simulink model "EV6_LUT_FourWheel_EV6Battery77p4kWh_PowerCorrected"  (R2024a)
settings: Solver=ode4  StartTime=0  StopTime=60  FixedStep=0.001  RelTol=1e-3
PreLoadFcn:
  | VSS_BICYCLE=Simulink.Variant('Dual=0');
  | VSS_DUAL=Simulink.Variant('Dual=1');
  | Dual=1;
  | load('DriveCycle2.mat')
PostLoadFcn:
  | if any(exist('dsrtsu_mdlpostloadfcn', 'file') ~= 0), dsrtsu_mdlpostloadfcn('Execute', bdroot); end
InitFcn:
  | , if any(exist('rtifpga_mdlclblib', 'file') ~= 0), rtifpga_mdlclblib('Init', bdroot); end,
  | , if any(exist('dsmpb_private', 'file') ~= 0), dsmpb_private('dsmpb_mdlclblib', 'Init', bdroot); end,
  | load('DriveCycle2.mat')
model workspace (MAT data in the model file):
  DiffRatio = 10.65
  EV6_2023_BattBranchCapacity_Ah = 55.5236728838
  EV6_2023_BattEnergy_kWh = 77.4
  EV6_2023_BattNominalVoltage_V = 697
  EV6_2023_BattNumCellsParallel = 2
  EV6_2023_BattNumCellsSeries = 192
  EV6_2023_BattOpenVoltCapBpts = [0 0.1 0.2 0.3 0.4 0.5 0.6 0.7 0.8 0.9 1]
  EV6_2023_BattOpenVoltTbl = [2.96762142548 3.40364281191 3.47417488548 3.54470541822 3.61523441014 3.68576186124 3.75628777151 3.82681214095 3.94527005036 4.07101207308 4.2120755254]
  EV6_2023_BattPackCapacity_Ah = 111.047345768
  EV6_2023_BattResistSocBpts = [0 0.2 0.4 0.6 0.8 1]
  EV6_2023_BattResistTbl = [0.0163620057716 0.0118174152018 0.00807187352333 0.00375663957972 0.00266904525531 0.00103635901355 0.0019014404175 0.0172368903217 0.0121226074867 0.00758541551769 0.00474065349228 0.00337561163613 ... (42 elements, 7x6)]
  EV6_2023_BattResistTempBpts = [243.1 253.1 263.1 273.1 283.1 298.1 313.1]
  EV6_2023_InitialPackOCV_V = 726.471714233
  EV6_2023_InitialSOC = 0.638878863672
  EV6_BattCellCapacity_Ah = 60.3
  EV6_BattInitialSOC = 0.638878863672
  EV6_BattOCV_Cell_V = [2.96762142548 3.40364281191 3.47417488548 3.54470541822 3.61523441014 3.68576186124 3.75628777151 3.82681214095 3.94527005036 4.07101207308 4.2120755254]
  EV6_BattOCV_SOC = [0 0.1 0.2 0.3 0.4 0.5 0.6 0.7 0.8 0.9 1]
  EV6_BattPackCapacity_Ah = 120.6
  EV6_BattParallelCells = 2
  EV6_BattResistanceSOC = [0 0.2 0.4 0.6 0.8 1]
  EV6_BattResistanceTable_Ohm = [0.0163620057716 0.0118174152018 0.00807187352333 0.00375663957972 0.00266904525531 0.00103635901355 0.0019014404175 0.0172368903217 0.0121226074867 0.00758541551769 0.00474065349228 0.00337561163613 ... (42 elements, 7x6)]
  EV6_BattResistanceTemp_K = [243.1 253.1 263.1 273.1 283.1 298.1 313.1]
  EV6_BattSeriesCells = 192
  EV6_FinalDriveRatio = 10.65
  EV6_TargetPackResistance_Ohm = 0.132763804608
  Gas = 0.383333333333
undefined symbols (not defined in the file): accel_bp_mps2, AccelCmd, ActTqLF_Nm_, ActTqLR_Nm_, ActTqRF_Nm_, ActTqRR_Nm_, BattChargeLimitMaxPwr, BattChargeLimitSocBpts, BattChargeLimitTbl, BattDischargeLimitSocBpts, BattDischargeLimitTbl, BattDischargeMaxPwr, BrakeMaxPrs, BrakeMaxTrq, ChassisDistCg2FrontAxle, ChassisDistCg2RearAxle, ChassisVehMass, CltchCmd, CoastDown, DecelCmd, DiscIntNeverNeededParam, EnvGravCnst, EnvPrs, EnvTemp, EV6_RegenTorqueGain, EV6_TractionTorqueGain, front_share_regen_3d, front_share_traction_3d, FuelSpecificGrav, GearCmd, h, InitStates, lgSw, limitedMCT, MCT, MtrEffSpdBpts, MtrEffTbl, MtrEffTrqBpts, MtrPwrMax, MtrTrqMax, out_1, pMCT, RealSimPara, Ref_speed, Ref_time, regen_torque_bp_Nm, speed_bp_kph, SteeringCmd, SupvsryCtrlRegenBrkCutOffTbl, SupvsryCtrlRegenSpdBpts, TestScnrioCycleNum, traction_torque_bp_Nm, US06, VEH
libraries: VSIGenLib x65, simulink x54, etargetslib x38, dsmpblib x24, vehdynlibtire x12, autolibshared x11, vehdynlibsuspension x7, vehdynlibtirecommon x7, autolibpowerinfoutils x6, autolibutils x5, autolibsharedcoupling x4, autolibmappedmotor x4
(part 9 of 19)

== system EV6_LUT_FourWheel_EV6Battery77p4kWh_PowerCorrected/Vehicle Under Test1/Vehicle/Vehicle Dynamics/Vehicle 14DOF/Suspension ==
  Steering : Inport
  Vehicle : Inport  Port=2
  Wheel : Inport  Port=3
  Double Wishbone Suspension : Subsystem  VariantControl=1
      mask Display: image('suspdw.png');
  Independent Mapped Front Suspension Mapped Solid Axle Rear Suspension : Subsystem  VariantControl=2
      mask Display: image([imread('suspindmap.png');imread('suspsamap.png')]);
  MacPherson Front Suspension Solid Axle Rear Suspension : Subsystem  VariantControl=3
      mask Display: image([imread('suspmacp.png');imread('suspsacoil.png')]);
  MacPherson Suspension : Subsystem  VariantControl=4
      mask Display: image('suspmacp.png');
  Mapped Suspension : Subsystem  VariantControl=5
      mask Display: image('suspindmap.png');
  Suspension : Outport  VectorParamsAs1DForOutWhenUnconnected=off

== system EV6_LUT_FourWheel_EV6Battery77p4kWh_PowerCorrected/Vehicle Under Test1/Vehicle/Vehicle Dynamics/Vehicle 14DOF/Vehicle ==
  Suspension : Inport
  Wind : Inport  Port=2
  Variant Subsystem : Subsystem  Variant=on  VariantControlMode=label  LabelModeActiveChoice=0
  VehFdbk : Outport  VectorParamsAs1DForOutWhenUnconnected=off
  wires:
  Suspension/1 -> Variant Subsystem/1(Suspension)
  Wind/1 -> Variant Subsystem/2(Wind)
  Variant Subsystem/1(VehFdbk) -> VehFdbk/1  "VehFdbk"

== system EV6_LUT_FourWheel_EV6Battery77p4kWh_PowerCorrected/Vehicle Under Test1/Vehicle/Vehicle Dynamics/Vehicle 14DOF/Vehicle Routing ==
  Veh : Inport
  Bus Selector10 : BusSelector  OutputSignals=BdyFrm.Cg.Vel.xdot,BdyFrm.Cg.Vel.ydot,BdyFrm.Cg.Vel.zdot  OutputAsBus=on
  Bus Selector2 : BusSelector  OutputSignals=InertFrm.Cg.Disp.X,InertFrm.Cg.Disp.Y,InertFrm.Cg.Disp.Z  OutputAsBus=on
  Bus Selector3 : BusSelector  OutputSignals=InertFrm.Cg.Vel.Xdot,InertFrm.Cg.Vel.Ydot,InertFrm.Cg.Vel.Zdot  OutputAsBus=on
  Bus Selector4 : BusSelector  OutputSignals=BdyFrm.Cg.Acc.ax,BdyFrm.Cg.Acc.ay,BdyFrm.Cg.Acc.az  OutputAsBus=on
  Bus Selector5 : BusSelector  OutputSignals=InertFrm.Cg.Ang.phi,InertFrm.Cg.Ang.theta,InertFrm.Cg.Ang.psi  OutputAsBus=on
  Bus Selector6 : BusSelector  OutputSignals=BdyFrm.Cg.AngVel.p,BdyFrm.Cg.AngVel.q,BdyFrm.Cg.AngVel.r  OutputAsBus=on
  Bus Selector7 : BusSelector  OutputSignals=InertFrm.Geom.Disp.X,InertFrm.Geom.Disp.Y,InertFrm.Geom.Disp.Z  OutputAsBus=on
  Bus Selector8 : BusSelector  OutputSignals=InertFrm.Geom.Vel.Xdot,InertFrm.Geom.Vel.Ydot,InertFrm.Geom.Vel.Zdot  OutputAsBus=on
  Bus Selector9 : BusSelector  OutputSignals=BdyFrm.Geom.Ang.Beta
  Bus to Vector{1..8} (8 alike) : BusToVector
  Cgxyzdot : Outport  VectorParamsAs1DForOutWhenUnconnected=off
  CgXYZ : Outport  Port=2  VectorParamsAs1DForOutWhenUnconnected=off
  CgXYZdot : Outport  Port=3  VectorParamsAs1DForOutWhenUnconnected=off
  angles : Outport  Port=4  VectorParamsAs1DForOutWhenUnconnected=off
  pqr : Outport  Port=5  VectorParamsAs1DForOutWhenUnconnected=off
  Cgaxyz : Outport  Port=6  VectorParamsAs1DForOutWhenUnconnected=off
  Beta : Outport  Port=7  VectorParamsAs1DForOutWhenUnconnected=off
  GeomXYZ : Outport  Port=8  VectorParamsAs1DForOutWhenUnconnected=off
  GeomXYZdot : Outport  Port=9  VectorParamsAs1DForOutWhenUnconnected=off
  wires:
  Veh/1 -> Bus Selector10/1, Bus Selector2/1, Bus Selector3/1, Bus Selector5/1, Bus Selector6/1, Bus Selector4/1, Bus Selector9/1, Bus Selector7/1, Bus Selector8/1
  Bus to Vector2/1 -> CgXYZdot/1
  Bus Selector7/1 -> Bus to Vector6/1
  Bus to Vector3/1 -> Cgaxyz/1
  Bus to Vector7/1 -> GeomXYZdot/1
  Bus Selector10/1 -> Bus to Vector8/1
  Bus Selector4/1 -> Bus to Vector3/1
  Bus Selector9/1 -> Beta/1  "<Beta>"
  Bus to Vector6/1 -> GeomXYZ/1
  Bus Selector8/1 -> Bus to Vector7/1
  Bus Selector2/1 -> Bus to Vector1/1
  Bus to Vector8/1 -> Cgxyzdot/1
  Bus to Vector4/1 -> angles/1
  Bus Selector6/1 -> Bus to Vector5/1
  Bus Selector5/1 -> Bus to Vector4/1
  Bus to Vector5/1 -> pqr/1
  Bus to Vector1/1 -> CgXYZ/1
  Bus Selector3/1 -> Bus to Vector2/1

== system EV6_LUT_FourWheel_EV6Battery77p4kWh_PowerCorrected/Vehicle Under Test1/Vehicle/Vehicle Dynamics/Vehicle 14DOF/Vehicle Routing1 ==
  Veh : Inport
  Bus Selector1 : BusSelector  OutputSignals=BdyFrm.Cg.Acc.xddot,BdyFrm.Cg.Acc.yddot,BdyFrm.Cg.Acc.zddot  OutputAsBus=on
  Bus Selector10 : BusSelector  OutputSignals=BdyFrm.Cg.Vel.xdot,BdyFrm.Cg.Vel.ydot,BdyFrm.Cg.Vel.zdot  OutputAsBus=on
  Bus Selector2 : BusSelector  OutputSignals=InertFrm.Cg.Disp.X,InertFrm.Cg.Disp.Y,InertFrm.Cg.Disp.Z  OutputAsBus=on
  Bus Selector3 : BusSelector  OutputSignals=InertFrm.Cg.Vel.Xdot,InertFrm.Cg.Vel.Ydot,InertFrm.Cg.Vel.Zdot  OutputAsBus=on
  Bus Selector4 : BusSelector  OutputSignals=BdyFrm.Cg.Acc.ax,BdyFrm.Cg.Acc.ay,BdyFrm.Cg.Acc.az  OutputAsBus=on
  Bus Selector5 : BusSelector  OutputSignals=InertFrm.Cg.Ang.phi,InertFrm.Cg.Ang.theta,InertFrm.Cg.Ang.psi  OutputAsBus=on
  Bus Selector6 : BusSelector  OutputSignals=BdyFrm.Cg.AngVel.p,BdyFrm.Cg.AngVel.q,BdyFrm.Cg.AngVel.r  OutputAsBus=on
  Bus Selector7 : BusSelector  OutputSignals=InertFrm.Geom.Disp.X,InertFrm.Geom.Disp.Y,InertFrm.Geom.Disp.Z  OutputAsBus=on
  Bus Selector8 : BusSelector  OutputSignals=InertFrm.Geom.Vel.Xdot,InertFrm.Geom.Vel.Ydot,InertFrm.Geom.Vel.Zdot  OutputAsBus=on
  Bus Selector9 : BusSelector  OutputSignals=BdyFrm.Geom.Ang.Beta
  Bus to Vector{1..9} (9 alike) : BusToVector
  Cgxyzdot : Outport  VectorParamsAs1DForOutWhenUnconnected=off
  CgXYZ : Outport  Port=2  VectorParamsAs1DForOutWhenUnconnected=off
  CgXYZdot : Outport  Port=3  VectorParamsAs1DForOutWhenUnconnected=off
  angles : Outport  Port=4  VectorParamsAs1DForOutWhenUnconnected=off
  pqr : Outport  Port=5  VectorParamsAs1DForOutWhenUnconnected=off
  Cgaxyz : Outport  Port=6  VectorParamsAs1DForOutWhenUnconnected=off
  Beta : Outport  Port=7  VectorParamsAs1DForOutWhenUnconnected=off
  GeomXYZ : Outport  Port=8  VectorParamsAs1DForOutWhenUnconnected=off
  GeomXYZdot : Outport  Port=9  VectorParamsAs1DForOutWhenUnconnected=off
  Cgxyzdotdot : Outport  Port=10  VectorParamsAs1DForOutWhenUnconnected=off
  wires:
  Bus Selector3/1 -> Bus to Vector2/1
  Bus to Vector1/1 -> CgXYZ/1
  Bus to Vector5/1 -> pqr/1
  Bus Selector5/1 -> Bus to Vector4/1
  Bus Selector6/1 -> Bus to Vector5/1
  Bus to Vector4/1 -> angles/1
  Bus to Vector8/1 -> Cgxyzdot/1
  Bus Selector2/1 -> Bus to Vector1/1
  Bus Selector8/1 -> Bus to Vector7/1
  Bus to Vector6/1 -> GeomXYZ/1
  Bus Selector9/1 -> Beta/1  "<Beta>"
  Bus Selector4/1 -> Bus to Vector3/1
  Bus Selector10/1 -> Bus to Vector8/1
  Bus to Vector7/1 -> GeomXYZdot/1
  Bus to Vector3/1 -> Cgaxyz/1
  Bus Selector7/1 -> Bus to Vector6/1
  Bus to Vector2/1 -> CgXYZdot/1
  Veh/1 -> Bus Selector8/1, Bus Selector7/1, Bus Selector9/1, Bus Selector4/1, Bus Selector6/1, Bus Selector5/1, Bus Selector3/1, Bus Selector2/1, Bus Selector10/1, Bus Selector1/1
  Bus Selector1/1 -> Bus to Vector9/1
  Bus to Vector9/1 -> Cgxyzdotdot/1

== system EV6_LUT_FourWheel_EV6Battery77p4kWh_PowerCorrected/Vehicle Under Test1/Vehicle/Vehicle Dynamics/Vehicle 14DOF/Wheel Routing ==
  Info : Inport
  Wheel : Inport  Port=2
  Bus Selector : BusSelector  OutputSignals=InertFrm.FrntAxl.Lft.Disp.Y,InertFrm.FrntAxl.Rght.Disp.Y,InertFrm.RearAxl.Lft.Disp.Y,InertFrm.RearAxl.Rght.Disp.Y
  Bus Selector1 : BusSelector  OutputSignals=InertFrm.FrntAxl.Lft.Disp.X,InertFrm.FrntAxl.Rght.Disp.X,InertFrm.RearAxl.Lft.Disp.X,InertFrm.RearAxl.Rght.Disp.X
  Bus Selector2 : BusSelector  OutputSignals=TireFrame.z,TireFrame.Omega,TireFrame.Kappa,TireFrame.Alpha
  Bus Selector3 : BusSelector  OutputSignals=InertFrm.FrntAxl.Lft.Disp.Z,InertFrm.FrntAxl.Rght.Disp.Z,InertFrm.RearAxl.Lft.Disp.Z,InertFrm.RearAxl.Rght.Disp.Z
  Bus Selector4 : BusSelector  OutputSignals=BdyFrm.FrntAxl.Lft.Disp.z,BdyFrm.FrntAxl.Rght.Disp.z,BdyFrm.RearAxl.Lft.Disp.z,BdyFrm.RearAxl.Rght.Disp.z
  Subtract : Sum  Inputs=-+-
  Vector Concatenate{1..4} (4 alike) : Concatenate  NumInputs=4
  Omega : Outport  PortDimensions=4  VectorParamsAs1DForOutWhenUnconnected=off
  Kappa : Outport  Port=2  PortDimensions=4  VectorParamsAs1DForOutWhenUnconnected=off
  Alpha : Outport  Port=3  PortDimensions=4  VectorParamsAs1DForOutWhenUnconnected=off
  XWheel : Outport  Port=4  Unit=m  VectorParamsAs1DForOutWhenUnconnected=off
  YWheel : Outport  Port=5  Unit=m  VectorParamsAs1DForOutWhenUnconnected=off
  ZWheel : Outport  Port=6  PortDimensions=4  VectorParamsAs1DForOutWhenUnconnected=off
  wires:
  Bus Selector4/2 -> Vector Concatenate4/2  "<z>"
  Bus Selector4/3 -> Vector Concatenate4/3  "<z>"
  Bus Selector4/4 -> Vector Concatenate4/4  "<z>"
  Bus Selector4/1 -> Vector Concatenate4/1  "<z>"
  Vector Concatenate4/1 -> Subtract/1
  Vector Concatenate3/1 -> Subtract/2
  Bus Selector3/1 -> Vector Concatenate3/1  "<Z>"
  Bus Selector3/4 -> Vector Concatenate3/4  "<Z>"
  Bus Selector3/3 -> Vector Concatenate3/3  "<Z>"
  Bus Selector3/2 -> Vector Concatenate3/2  "<Z>"
  Info/1 -> Bus Selector/1, Bus Selector3/1, Bus Selector4/1, Bus Selector1/1
  Subtract/1 -> ZWheel/1
  Wheel/1 -> Bus Selector2/1
  Bus Selector2/4 -> Alpha/1  "<Alpha>"
  Bus Selector2/3 -> Kappa/1  "<Kappa>"
  Bus Selector2/2 -> Omega/1  "<Omega>"
  Bus Selector2/1 -> Subtract/3  "<z>"
  Vector Concatenate2/1 -> XWheel/1
  Bus Selector1/1 -> Vector Concatenate2/1  "<X>"
  Vector Concatenate1/1 -> YWheel/1
  Bus Selector/2 -> Vector Concatenate1/2  "<Y>"
  Bus Selector/3 -> Vector Concatenate1/3  "<Y>"
  Bus Selector1/2 -> Vector Concatenate2/2  "<X>"
  Bus Selector/4 -> Vector Concatenate1/4  "<Y>"
  Bus Selector1/3 -> Vector Concatenate2/3  "<X>"
  Bus Selector/1 -> Vector Concatenate1/1  "<Y>"
  Bus Selector1/4 -> Vector Concatenate2/4  "<X>"

== system EV6_LUT_FourWheel_EV6Battery77p4kWh_PowerCorrected/Vehicle Under Test1/Vehicle/Vehicle Dynamics/Vehicle 14DOF/Wheel Routing1 ==
  Info : Inport
  Wheel : Inport  Port=2
  Bus Selector : BusSelector  OutputSignals=InertFrm.FrntAxl.Lft.Disp.Y,InertFrm.FrntAxl.Rght.Disp.Y,InertFrm.RearAxl.Lft.Disp.Y,InertFrm.RearAxl.Rght.Disp.Y
  Bus Selector1 : BusSelector  OutputSignals=InertFrm.FrntAxl.Lft.Disp.X,InertFrm.FrntAxl.Rght.Disp.X,InertFrm.RearAxl.Lft.Disp.X,InertFrm.RearAxl.Rght.Disp.X
  Bus Selector2 : BusSelector  OutputSignals=TireFrame.z,TireFrame.Omega,TireFrame.Kappa,TireFrame.Alpha
  Bus Selector3 : BusSelector  OutputSignals=InertFrm.FrntAxl.Lft.Disp.Z,InertFrm.FrntAxl.Rght.Disp.Z,InertFrm.RearAxl.Lft.Disp.Z,InertFrm.RearAxl.Rght.Disp.Z
  Bus Selector4 : BusSelector  OutputSignals=BdyFrm.FrntAxl.Lft.Disp.z,BdyFrm.FrntAxl.Rght.Disp.z,BdyFrm.RearAxl.Lft.Disp.z,BdyFrm.RearAxl.Rght.Disp.z
  Scope : Scope
  Scope1 : Scope
  Subtract : Sum  Inputs=-+-
  Vector Concatenate{1..4} (4 alike) : Concatenate  NumInputs=4
  Omega : Outport  PortDimensions=4  VectorParamsAs1DForOutWhenUnconnected=off
  Kappa : Outport  Port=2  PortDimensions=4  VectorParamsAs1DForOutWhenUnconnected=off
  Alpha : Outport  Port=3  PortDimensions=4  VectorParamsAs1DForOutWhenUnconnected=off
  XWheel : Outport  Port=4  Unit=m  VectorParamsAs1DForOutWhenUnconnected=off
  YWheel : Outport  Port=5  Unit=m  VectorParamsAs1DForOutWhenUnconnected=off
  ZWheel : Outport  Port=6  PortDimensions=4  VectorParamsAs1DForOutWhenUnconnected=off
  wires:
  Bus Selector1/4 -> Vector Concatenate2/4  "<X>"
  Bus Selector/1 -> Vector Concatenate1/1  "<Y>"
  Bus Selector1/3 -> Vector Concatenate2/3  "<X>"
  Bus Selector/4 -> Vector Concatenate1/4  "<Y>"
  Bus Selector1/2 -> Vector Concatenate2/2  "<X>"
  Bus Selector/3 -> Vector Concatenate1/3  "<Y>"
  Bus Selector/2 -> Vector Concatenate1/2  "<Y>"
  Vector Concatenate1/1 -> YWheel/1
  Bus Selector1/1 -> Vector Concatenate2/1  "<X>"
  Vector Concatenate2/1 -> XWheel/1
  Bus Selector2/1 -> Subtract/3, Scope1/1  "<z>"
  Bus Selector2/2 -> Omega/1, Scope/1  "<Omega>"
  Bus Selector2/3 -> Kappa/1  "<Kappa>"
  Bus Selector2/4 -> Alpha/1  "<Alpha>"
  Wheel/1 -> Bus Selector2/1
  Subtract/1 -> ZWheel/1
  Info/1 -> Bus Selector1/1, Bus Selector4/1, Bus Selector3/1, Bus Selector/1
  Bus Selector3/2 -> Vector Concatenate3/2  "<Z>"
  Bus Selector3/3 -> Vector Concatenate3/3  "<Z>"
  Bus Selector3/4 -> Vector Concatenate3/4  "<Z>"
  Bus Selector3/1 -> Vector Concatenate3/1  "<Z>"
  Vector Concatenate3/1 -> Subtract/2
  Vector Concatenate4/1 -> Subtract/1
  Bus Selector4/1 -> Vector Concatenate4/1  "<z>"
  Bus Selector4/4 -> Vector Concatenate4/4  "<z>"
  Bus Selector4/3 -> Vector Concatenate4/3  "<z>"
  Bus Selector4/2 -> Vector Concatenate4/2  "<z>"

== system EV6_LUT_FourWheel_EV6Battery77p4kWh_PowerCorrected/Vehicle Under Test1/Vehicle/Vehicle Dynamics/Vehicle 14DOF/Wheels and Tires ==
  Suspension : Inport
  Axle Torque : Inport  Port=2
  Brake Press : Inport  Port=3  Unit=Pa
  Ground Input : Inport  Port=4
  Friction : Inport  Port=5  PortDimensions=4
  Bus Selector1 : BusSelector  OutputSignals=Whl.Ang,Whl.F,Whl.AngVel,Whl.xdot,Whl.ydot
  Constant3 : Constant  Value=zeros(4,1)
  Cont LPF : autolibutils/Cont LPF  wc=100*2*pi  AbsoluteTolerance=auto  aMode=2
  Cont LPF1 : autolibutils/Cont LPF  wc=100*2*pi  AbsoluteTolerance=auto  aMode=2
  Manual Switch6 : ManualSwitch
  Matrix Concatenate : Concatenate  NumInputs=3  Mode=Multidimensional array
  Reshape1 : Reshape
  Reshape2 : Reshape
  Saturation : Saturate  UpperLimit=10*9.81*2040  LowerLimit=-10*9.81*2040  ZeroCross=off
  Scope : Scope
  Scope1 : Scope
  Scope2 : Scope
  Selector : Selector  NumberOfDimensions=2  InputPortWidth=3  IndexOptions=Index vector (dialog),Select all  Indices=[3],1  OutputSizes=1,1
  Selector1 : Selector  NumberOfDimensions=2  InputPortWidth=1  IndexOptions=Index vector (dialog),Select all  Indices=[3],1  OutputSizes=1,1
  Selector2 : Selector  NumberOfDimensions=2  InputPortWidth=3  IndexOptions=Index vector (dialog),Select all  Indices=3,1  OutputSizes=1,1
  Selector3 : Selector  NumberOfDimensions=2  InputPortWidth=3  IndexOptions=Index vector (dialog),Select all  Indices=1,1  OutputSizes=1,1
  Terminator{,1,3..5} (5 alike) : Terminator
  VDBS : Subsystem  VariantControl=0
  Wheels : Outport  VectorParamsAs1DForOutWhenUnconnected=off
  wires:
  Cont LPF1/1 -> Selector2/1, Selector3/1
  Cont LPF/1 -> Scope/1, Saturation/1
  Friction/1 -> VDBS/9(Friction)
  Brake Press/1 -> VDBS/4(BrkPrs)
  Reshape1/1 -> VDBS/6(r)
  Bus Selector1/3 -> Selector1/1  "<AngVel>"
  Reshape2/1 -> Cont LPF/1
  VDBS/6(SuspWhlPz) -> Terminator5/1  "z"
  Bus Selector1/5 -> Matrix Concatenate/2  "<ydot>"
  Bus Selector1/4 -> Matrix Concatenate/1  "<xdot>"
  Suspension/1 -> Bus Selector1/1
  Selector3/1 -> Manual Switch6/2  "Camber Angles"
  Bus Selector1/1 -> Cont LPF1/1  "<Ang>"
  VDBS/7(SuspWhlVz) -> Matrix Concatenate/3  "zdot"
  Ground Input/1 -> VDBS/8(Ground Level)
  Saturation/1 -> Scope1/1, VDBS/5(Fz)
  Selector/1 -> Reshape2/1
  Manual Switch6/1 -> VDBS/2(CamberAng)  "Camber Angles"
  Constant3/1 -> Manual Switch6/1
  Selector2/1 -> VDBS/1(WheelAng)  "Wheel Angles"
  Axle Torque/1 -> Scope2/1, VDBS/3(AxleTrq)
  Matrix Concatenate/1 -> VDBS/7(VehVel)
  Selector1/1 -> Reshape1/1
  VDBS/5(Mz) -> Terminator4/1
  VDBS/4(Omega) -> Terminator3/1
  VDBS/3(RearAxlF) -> Terminator1/1
  VDBS/2(FrntAxlF) -> Terminator/1
  Bus Selector1/2 -> Selector/1  "<F>"
  VDBS/1(Wheels) -> Wheels/1  "Wheels"

== system EV6_LUT_FourWheel_EV6Battery77p4kWh_PowerCorrected/Vehicle Under Test1/Vehicle/Vehicle Dynamics/Vehicle 7DOF/Brake Pressure ==
  BrkReq : Inport
  Bus Creator1 : BusCreator  Inputs=2
  Gain : Gain  Gain=BrakeMaxPrs
  Gain{1..4} (4 alike) : Gain  Gain=0.5
  Saturation{,1..3} (4 alike) : Saturate  UpperLimit=BrakeMaxPrs  LowerLimit=0  ZeroCross=off
  Signal Specification : SignalSpecification  Unit=Pa
  Terminator : Terminator
  Vector Concatenate2 : Concatenate  NumInputs=4
  BrakePrs : Outport  Unit=Pa
  wires:
  Saturation3/1 -> Vector Concatenate2/4
  Saturation2/1 -> Vector Concatenate2/3
  Saturation1/1 -> Vector Concatenate2/2
  Saturation/1 -> Vector Concatenate2/1
  Vector Concatenate2/1 -> BrakePrs/1
  Gain4/1 -> Saturation3/1, Saturation2/1
  Gain3/1 -> Saturation1/1, Saturation/1
  Gain2/1 -> Gain3/1
  Gain1/1 -> Gain4/1
  Bus Creator1/1 -> Terminator/1  "WhlBrk"
  Signal Specification/1 -> Bus Creator1/2, Gain1/1, Gain2/1  "BrkPrs"
  Gain/1 -> Signal Specification/1
  BrkReq/1 -> Bus Creator1/1, Gain/1  "BrkReq"

== system EV6_LUT_FourWheel_EV6Battery77p4kWh_PowerCorrected/Vehicle Under Test1/Vehicle/Vehicle Dynamics/Vehicle 7DOF/Longitudinal Wheels 4DOF ==
  WhlAng : Inport
  AxlTrq : Inport  Port=2
  BrkPrs : Inport  Port=3
  Gnd : Inport  Port=4  PortDimensions=4
  lam_mu : Inport  Port=5  PortDimensions=4
  VehFdbk : Inport  Port=6
  Axle Forces : Subsystem  Variant=on  VariantControlMode=label  LabelModeActiveChoice=1
  Bus Selector5 : BusSelector  OutputSignals=BdyFrm.Cg.AngVel.r
  Constant : vehdynlibtirecommon/Constant  const=220000  numWheels=4
  Constant3 : vehdynlibtirecommon/Constant  const=0  numWheels=4
  Terminator2 : Terminator
  Tire2Veh : Subsystem
  Tires : Subsystem
  Veh2Tire : Subsystem
  Velocity and Vertical Load : Subsystem  Variant=on  VariantControlMode=label  LabelModeActiveChoice=1
  Wheel Angles : Subsystem
  FrntAxlF : Outport  Unit=N  VectorParamsAs1DForOutWhenUnconnected=off
  RearAxlF : Outport  Port=2  Unit=N  VectorParamsAs1DForOutWhenUnconnected=off
  Omega : Outport  Port=3  VectorParamsAs1DForOutWhenUnconnected=off
  Kappa : Outport  Port=4  VectorParamsAs1DForOutWhenUnconnected=off
  Alpha : Outport  Port=5  VectorParamsAs1DForOutWhenUnconnected=off
  zAxle : Outport  Port=6  VectorParamsAs1DForOutWhenUnconnected=off
  wires:
  Tire2Veh/6(Alpha) -> Alpha/1
  Tire2Veh/5(Kappa) -> Kappa/1
  Tire2Veh/4(Omega) -> Omega/1
  Tire2Veh/3(z) -> zAxle/1
  Tire2Veh/2(FwR) -> Axle Forces/2(R)
  Tire2Veh/1(FwF) -> Axle Forces/1(F)
  Axle Forces/2(RearAxlF) -> RearAxlF/1
  Axle Forces/1(FrntAxlF) -> FrntAxlF/1
  Velocity and Vertical Load/1(VehVel) -> Veh2Tire/4(VehVel)
  Velocity and Vertical Load/2(Fz) -> Tires/8(Fz)
  Veh2Tire/5(psidot) -> Tires/5(r)
  Veh2Tire/4(ydotAxle) -> Tires/4(Vy)  "Vy"
  WhlAng/1 -> Wheel Angles/1(WheelAng)  "FrontWheelAngles"
  Veh2Tire/6(zdotAxle) -> Terminator2/1
  Bus Selector5/1 -> Veh2Tire/3(r)  "<r>"
  BrkPrs/1 -> Veh2Tire/2(BrkPrs)
  Veh2Tire/2(P) -> Tires/2(BrkPrs)
  Veh2Tire/1(T) -> Tires/1(AxlTrq)
  AxlTrq/1 -> Veh2Tire/1(AxlTrq)
  VehFdbk/1 -> Velocity and Vertical Load/1(VehFdbk), Bus Selector5/1
  Gnd/1 -> Tires/10(Gnd)
  Veh2Tire/3(xdotAxle) -> Tires/3(Vx)  "Vx"
  Constant3/1 -> Tires/6(Camber), Wheel Angles/2(Camber)
  Constant/1 -> Tires/7(TirePrs)
  lam_mu/1 -> Tires/9(lam_mu)
  Tires/1(Wheel) -> Tire2Veh/1(Wheel)
  Wheel Angles/1(WhlAngB) -> Veh2Tire/5(WhlAng)

== system EV6_LUT_FourWheel_EV6Battery77p4kWh_PowerCorrected/Vehicle Under Test1/Vehicle/Vehicle Dynamics/Vehicle 7DOF/RototestDummy ==
  Bus Creator1 : BusCreator  Inputs=ActTqLF_Nm_,ActTqRF_Nm_,ActTqLR_Nm_,ActTqRR_Nm_
  Bus Creator2 : BusCreator  Inputs=Car Trq_T2WFL,Car Trq_T2WFR,Car Trq_T2WRL,Car Trq_T2WRR
  Bus Creator3 : BusCreator  Inputs=1
  Bus Creator4 : BusCreator  Inputs=1
  Bus Selector14 : BusSelector  OutputSignals=VehSpd
  Bus Selector15 : BusSelector  OutputSignals=TireFrame.Fx
  Constant{1..14} (14 alike) : Constant  Value=0
  Vector Concatenate3 : Concatenate  NumInputs=4
  CarTrqT2W : Outport
  AxleTrq : Outport  Port=2
  BrakePressed_flag : Outport  Port=3
  <VehSpd> : Outport  Port=4
  <Fx> : Outport  Port=5
  wires:
  Bus Selector15/1 -> <Fx>/1  "<Fx>"
  Constant5/1 -> BrakePressed_flag/1  "BrakePressed_flag"
  Bus Selector14/1 -> <VehSpd>/1  "<VehSpd>"
  Bus Creator2/1 -> CarTrqT2W/1  "CarTrqT2W"
  Constant12/1 -> Bus Creator2/2  "CarTrq_T2WFR"
  Constant7/1 -> Bus Creator1/2  "ActTqRF_Nm_"
  Constant11/1 -> Bus Creator2/1  "CarTrq_T2WFL"
  Constant8/1 -> Bus Creator1/3  "ActTqLR_Nm_"
  Constant1/1 -> Vector Concatenate3/1
  Constant6/1 -> Bus Creator1/1  "ActTqLF_Nm_"
  Constant14/1 -> Bus Creator2/4  "CarTrq_T2WRR"
  Constant2/1 -> Vector Concatenate3/2
  Constant3/1 -> Vector Concatenate3/3
  Vector Concatenate3/1 -> Bus Creator4/1  "Fx"
  Bus Creator3/1 -> Bus Selector15/1
  Constant4/1 -> Vector Concatenate3/4
  Constant13/1 -> Bus Creator2/3  "CarTrq_T2WRL"
  Constant9/1 -> Bus Creator1/4  "ActTqRR_Nm_"
  Bus Creator1/1 -> AxleTrq/1  "AxleTrq"
  Bus Creator4/1 -> Bus Creator3/1  "TireFrame"
  Constant10/1 -> Bus Selector14/1  "VehSpd"

== system EV6_LUT_FourWheel_EV6Battery77p4kWh_PowerCorrected/Vehicle Under Test1/Vehicle/Vehicle Dynamics/Vehicle 7DOF/Steering ==
  SteeringCmd : Inport
  Ground : Ground
  Kinematic Steering : vehdynlibsteering/Kinematic Steering  StrgType=Ackerman  StrgRatioType=Constant  Loc=Front  NrmlFctr=1  TrckWdth=1.9  WhlBase=ChassisDistCg2FrontAxle+ChassisDistCg2RearAxle  Db=0  StrgRng=3*pi  StrgAngBpts="[-6.2832   -5.0265   -3.7699   -2.5133   -1.2566         0    1.2566    2.5133    3.7699    5.0265    6.2832]"  StrgRatioTbl=|  StrgRatio=18  PctAckIn=off  PctAck=100  PctAckTbl=ones(1,11)*100  StrgArmLngth=0.1  RckCsLngth=0.5  TieRodLngth=0.248  D=0.2  PnnRadius=0.0057  PnnRadiusTbl="[0.0055    0.0055    0.0056    0.0057    0.0058    0.0057    0.0057    0.0057    0.0056    0.0055    0.0055]"  RodLngth=0.1  ParaArmLngth=0.9  aMode=2
      | [13.5000   13.3750   13.2500   13.1250   13.0000   13.0000   13.0000   13.1250   13.2500   13.3750   13.5000
      | ]
  Terminator1 : Terminator
  Vector Concatenate : Concatenate
  Vector Concatenate1 : Concatenate
  Vector Concatenate2 : Concatenate
  WhlAng : Outport  Unit=rad
  wires:
  SteeringCmd/1 -> Kinematic Steering/1
  Kinematic Steering/3 -> Vector Concatenate/2
  Ground/1 -> Vector Concatenate1/1, Vector Concatenate1/2
  Vector Concatenate/1 -> Vector Concatenate2/1  "FrontWheelAngles"
  Vector Concatenate1/1 -> Vector Concatenate2/2  "RearWheelAngles"
  Kinematic Steering/2 -> Vector Concatenate/1
  Vector Concatenate2/1 -> WhlAng/1
  Kinematic Steering/1 -> Terminator1/1

== system EV6_LUT_FourWheel_EV6Battery77p4kWh_PowerCorrected/Vehicle Under Test1/Vehicle/Vehicle Dynamics/Vehicle 7DOF/Subsystem4 ==
  Cgxyzdot : Inport
  CgXYZ : Inport  Port=2
  CgXYZdot : Inport  Port=3
  angles : Inport  Port=4
  pqr : Inport  Port=5
  Cgaxyz : Inport  Port=6
  Beta : Inport  Port=7
  GeomXYZ : Inport  Port=8
  GeomXYZdot : Inport  Port=9
  Omega : Inport  Port=10
  Kappa : Inport  Port=11
  Alpha : Inport  Port=12
  XWheel : Inport  Port=13
  YWheel : Inport  Port=14
  dzWheel : Inport  Port=15
  Bus Creator : BusCreator  Inputs=26
  Bus Creator3 : BusCreator  Inputs=6
  Demux{,1..7} (8 alike) : Demux  Outputs=3
  Subsystem : Subsystem
  Chassis : Outport  VectorParamsAs1DForOutWhenUnconnected=off
  Wheels : Outport  Port=2  VectorParamsAs1DForOutWhenUnconnected=off
  wires:
  Subsystem/1(VehSpd) -> Bus Creator/26  "VehSpd"
  Demux7/3 -> Bus Creator/25  "GeomZdot"
  Demux7/2 -> Bus Creator/24  "GeomYdot"
  Demux7/1 -> Bus Creator/23  "GeomXdot"
  Demux6/3 -> Bus Creator/22  "GeomZ"
  Demux6/2 -> Bus Creator/21  "GeomY"
  Demux6/1 -> Bus Creator/20  "GeomX"
  Beta/1 -> Bus Creator/19  "Beta"
  Demux5/3 -> Bus Creator/18  "az"
  Demux5/2 -> Bus Creator/17  "ay"
  Demux5/1 -> Bus Creator/16  "ax"
  Demux4/3 -> Bus Creator/15  "r"
  Demux4/2 -> Bus Creator/14  "q"
  Demux4/1 -> Bus Creator/13  "p"
  Demux3/3 -> Bus Creator/12  "psi"
  Demux3/2 -> Bus Creator/11  "theta"
  Demux3/1 -> Bus Creator/10  "phi"
  Demux2/3 -> Bus Creator/9  "Zdot"
  Demux2/2 -> Bus Creator/8  "Ydot"
  Demux2/1 -> Bus Creator/7  "Xdot"
  Demux1/3 -> Bus Creator/6  "Z"
  Demux1/2 -> Bus Creator/5  "Y"
  Demux1/1 -> Bus Creator/4  "X"
  Demux/3 -> Bus Creator/3  "zdot"
  Demux/2 -> Bus Creator/2  "ydot"
  Demux/1 -> Bus Creator/1  "xdot"
  GeomXYZ/1 -> Demux6/1
  GeomXYZdot/1 -> Demux7/1
  Cgaxyz/1 -> Demux5/1
  pqr/1 -> Demux4/1
  angles/1 -> Demux3/1, Subsystem/2(angles)
  CgXYZdot/1 -> Demux2/1, Subsystem/1(CgXYZdot)
  CgXYZ/1 -> Demux1/1
  Cgxyzdot/1 -> Demux/1
  Alpha/1 -> Bus Creator3/2  "Alpha"
  XWheel/1 -> Bus Creator3/4  "XWheel"
  YWheel/1 -> Bus Creator3/5  "YWheel"
  Bus Creator3/1 -> Wheels/1  "Wheels"
  Kappa/1 -> Bus Creator3/1  "Kappa"
  dzWheel/1 -> Bus Creator3/6  "dZWheel"
  Omega/1 -> Bus Creator3/3  "Omega"
  Bus Creator/1 -> Chassis/1  "Chassis"

== system EV6_LUT_FourWheel_EV6Battery77p4kWh_PowerCorrected/Vehicle Under Test1/Vehicle/Vehicle Dynamics/Vehicle 7DOF/Vehicle Body 3DOF External Longitudinal Wheels ==
  WhlAng : Inport
  "FwF " : Inport  Port=2
  "FwR " : Inport  Port=3
  WindXYZ : Inport  Port=4
  Friction : Inport  Port=5  Unit=1  PortDimensions=4
  Bicycle : Subsystem  VariantControl=0
  Dual : Subsystem  VariantControl=1
  " Info" : Outport  VectorParamsAs1DForOutWhenUnconnected=off
  " XWheel" : Outport  Port=2  VectorParamsAs1DForOutWhenUnconnected=off
  " YWheel" : Outport  Port=3  VectorParamsAs1DForOutWhenUnconnected=off

== system EV6_LUT_FourWheel_EV6Battery77p4kWh_PowerCorrected/Vehicle Under Test1/Vehicle/Vehicle Dynamics/Vehicle Longitudinal/Brake Pressure ==
  BrkReq : Inport
  Bus Creator1 : BusCreator  Inputs=2
  Gain : Gain  Gain=BrakeMaxPrs
  Gain{1..4} (4 alike) : Gain  Gain=0.5
  Saturation{,1..3} (4 alike) : Saturate  UpperLimit=BrakeMaxPrs  LowerLimit=0  ZeroCross=off
  Signal Specification : SignalSpecification  Unit=Pa
  Terminator : Terminator
  Vector Concatenate2 : Concatenate  NumInputs=4
  BrakePrs : Outport  Unit=Pa
  wires:
  Saturation3/1 -> Vector Concatenate2/4
  Saturation2/1 -> Vector Concatenate2/3
  Saturation1/1 -> Vector Concatenate2/2
  Saturation/1 -> Vector Concatenate2/1
  Vector Concatenate2/1 -> BrakePrs/1
  Gain4/1 -> Saturation3/1, Saturation2/1
  Gain3/1 -> Saturation1/1, Saturation/1
  Gain2/1 -> Gain3/1
  Gain1/1 -> Gain4/1
  Bus Creator1/1 -> Terminator/1  "WhlBrk"
  Signal Specification/1 -> Bus Creator1/2, Gain1/1, Gain2/1  "BrkPrs"
  Gain/1 -> Signal Specification/1
  BrkReq/1 -> Bus Creator1/1, Gain/1  "BrkReq"

== system EV6_LUT_FourWheel_EV6Battery77p4kWh_PowerCorrected/Vehicle Under Test1/Vehicle/Vehicle Dynamics/Vehicle Longitudinal/Longitudinal Wheels ==
  BrkPrs : Inport
  AxleTorq : Inport  Port=2
  Bus Creator : BusCreator  Inputs=3
  Bus Selector : BusSelector  OutputSignals=WhlRearInfo,Omega3,Omega4
  Bus Selector1 : BusSelector  OutputSignals=WhlFrontInfo,Omega1,Omega2
  Front Diff Wheels : Subsystem
  Rear Wheels : Subsystem
  Vector Concatenate : Concatenate  NumInputs=4
  FrontAxle : PMIOPort  Side=Right
  RearAxle : PMIOPort  Port=2  Side=Right
  Whl : Outport
  wires:
  Vector Concatenate/1 -> Bus Creator/3  "Omega"
  Bus Selector/1 -> Bus Creator/2  "<WhlRearInfo>"
  Bus Selector/3 -> Vector Concatenate/4  "<Omega4>"
  Bus Selector1/3 -> Vector Concatenate/2  "<Omega2>"
  Bus Selector1/2 -> Vector Concatenate/1  "<Omega1>"
  Bus Selector1/1 -> Bus Creator/1  "<WhlFrontInfo>"
  Bus Selector/2 -> Vector Concatenate/3  "<Omega3>"
  AxleTorq/1 -> Front Diff Wheels/2(AxleTorq)
  BrkPrs/1 -> Rear Wheels/1(BrkPrs), Front Diff Wheels/1(BrkPrs)
  Bus Creator/1 -> Whl/1  "Whl"
  Front Diff Wheels/1(Info) -> Bus Selector1/1  "WhlFrontInfo"
  Rear Wheels/1(Info) -> Bus Selector/1  "WhlRearInfo"
  connections:
  Front Diff Wheels/RConn1 -- FrontAxle/RConn1
  RearAxle/RConn1 -- Rear Wheels/RConn1

== system EV6_LUT_FourWheel_EV6Battery77p4kWh_PowerCorrected/Vehicle Under Test1/Vehicle/Vehicle Dynamics/Vehicle Longitudinal/RototestDummy ==
  Bus Creator1 : BusCreator  Inputs=ActTqLF_Nm_,ActTqRF_Nm_,ActTqLR_Nm_,ActTqRR_Nm_
  Bus Creator2 : BusCreator  Inputs=Car Trq_T2WFL,Car Trq_T2WFR,Car Trq_T2WRL,Car Trq_T2WRR
  Bus Creator3 : BusCreator  Inputs=1
  Bus Creator4 : BusCreator  Inputs=1
  Bus Selector14 : BusSelector  OutputSignals=VehSpd
  Bus Selector15 : BusSelector  OutputSignals=TireFrame.Fx
  Constant{1..14} (14 alike) : Constant  Value=0
  Vector Concatenate3 : Concatenate  NumInputs=4
  CarTrqT2W : Outport
  AxleTrq : Outport  Port=2
  BrakePressed_flag : Outport  Port=3
  <VehSpd> : Outport  Port=4
  <Fx> : Outport  Port=5
  wires:
  Bus Selector15/1 -> <Fx>/1  "<Fx>"
  Constant5/1 -> BrakePressed_flag/1  "BrakePressed_flag"
  Bus Selector14/1 -> <VehSpd>/1  "<VehSpd>"
  Bus Creator2/1 -> CarTrqT2W/1  "CarTrqT2W"
  Constant12/1 -> Bus Creator2/2  "CarTrq_T2WFR"
  Constant7/1 -> Bus Creator1/2  "ActTqRF_Nm_"
  Constant11/1 -> Bus Creator2/1  "CarTrq_T2WFL"
  Constant8/1 -> Bus Creator1/3  "ActTqLR_Nm_"
  Constant1/1 -> Vector Concatenate3/1
  Constant6/1 -> Bus Creator1/1  "ActTqLF_Nm_"
  Constant14/1 -> Bus Creator2/4  "CarTrq_T2WRR"
  Constant2/1 -> Vector Concatenate3/2
  Constant3/1 -> Vector Concatenate3/3
  Vector Concatenate3/1 -> Bus Creator4/1  "Fx"
  Bus Creator3/1 -> Bus Selector15/1
  Constant4/1 -> Vector Concatenate3/4
  Constant13/1 -> Bus Creator2/3  "CarTrq_T2WRL"
  Constant9/1 -> Bus Creator1/4  "ActTqRR_Nm_"
  Bus Creator1/1 -> AxleTrq/1  "AxleTrq"
  Bus Creator4/1 -> Bus Creator3/1  "TireFrame"
  Constant10/1 -> Bus Selector14/1  "VehSpd"

== system EV6_LUT_FourWheel_EV6Battery77p4kWh_PowerCorrected/Vehicle Under Test1/Vehicle/Vehicle Dynamics/Vehicle Longitudinal/Vehicle Body ==
  RoadGrade : Inport
  WindX : Inport  Port=2
  Logitudinal Vehicle Body : Subsystem
  Subsystem1 : Subsystem
      mask Display: disp('')
  FrontAxle : PMIOPort  Side=Left
  RearDiff : PMIOPort  Port=2  Side=Left
  Chassis : Outport
  wires:
  WindX/1 -> Logitudinal Vehicle Body/2(WindVel)
  RoadGrade/1 -> Logitudinal Vehicle Body/1(RoadGrade)
  Subsystem1/1(ChassisPlant) -> Chassis/1
  Logitudinal Vehicle Body/4(RearAxleFrc) -> Subsystem1/4(RearAxleFrc)
  Logitudinal Vehicle Body/3(FrontAxleFrc) -> Subsystem1/3(FrontAxleFrc)
  Logitudinal Vehicle Body/2(VehDist) -> Subsystem1/2(VehDist)
  Logitudinal Vehicle Body/1(VehSpd) -> Subsystem1/1(VehSpd)
  connections:
  FrontAxle/RConn1 -- Logitudinal Vehicle Body/LConn1
  RearDiff/RConn1 -- Logitudinal Vehicle Body/LConn2

== system EV6_LUT_FourWheel_EV6Battery77p4kWh_PowerCorrected/Vehicle Under Test1/Vehicle/Actuation and Outputs/MOOG Brake Actuator/ CAN Settings/ CAN diagnostic Counter ==
  RX Counter : Inport
  Compare To Constant3 : simulink/Logic and Bit Operations/Compare To Constant  relop=<=  const=TimeOutDuration  OutDataTypeStr=boolean
  Memory2 : Memory  InheritSampleTime=on
  Relational Operator2 : RelationalOperator  Operator=~=  OutDataTypeStr=boolean  InputSameDT=off
  Timer : Subsystem
  CommsOKFlag : Outport
  wires:
  Compare To Constant3/1 -> CommsOKFlag/1
  Memory2/1 -> Relational Operator2/2
  RX Counter/1 -> Memory2/1, Relational Operator2/1
  Timer/1(Timer) -> Compare To Constant3/1
  Relational Operator2/1 -> Timer/1(Reset)

== system EV6_LUT_FourWheel_EV6Battery77p4kWh_PowerCorrected/Vehicle Under Test1/Vehicle/Actuation and Outputs/MOOG Brake Actuator/MOOG Interface/Max Stop Adjustment ==
  In1 : Inport
  Enable : EnablePort
  MaxStopOffset : Constant  Value=-5500
  Sum3 : Sum  Inputs=|++
  Out1 : Outport  InitialOutput=[0]
  wires:
  Sum3/1 -> Out1/1
  In1/1 -> Sum3/1
  MaxStopOffset/1 -> Sum3/2

== system EV6_LUT_FourWheel_EV6Battery77p4kWh_PowerCorrected/Vehicle Under Test1/Vehicle/Actuation and Outputs/MOOG Brake Actuator/MOOG Interface/Min Stop Adjustment ==
  In1 : Inport
  Enable : EnablePort
  MinStopOffset : Constant  Value=3500
  Sum3 : Sum  Inputs=|++
  Out1 : Outport  InitialOutput=[0]
  wires:
  MinStopOffset/1 -> Sum3/2
  Sum3/1 -> Out1/1
  In1/1 -> Sum3/1

== system EV6_LUT_FourWheel_EV6Battery77p4kWh_PowerCorrected/Vehicle Under Test1/Vehicle/Actuation and Outputs/MOOG Brake Actuator/MOOG Interface/Rising edge ==
  In : Inport
  Memory : Memory  InheritSampleTime=on
  Sum3 : Sum  Inputs=|+-
  Out : Outport
  wires:
  Sum3/1 -> Out/1
  Memory/1 -> Sum3/2
  In/1 -> Sum3/1, Memory/1

== system EV6_LUT_FourWheel_EV6Battery77p4kWh_PowerCorrected/Vehicle Under Test1/Vehicle/Actuation and Outputs/MOOG Brake Actuator/MOOG Interface/Rising edge1 ==
  In : Inport
  Memory : Memory  InheritSampleTime=on
  Sum3 : Sum  Inputs=|+-
  Out : Outport
  wires:
  Sum3/1 -> Out/1
  Memory/1 -> Sum3/2
  In/1 -> Sum3/1, Memory/1

== system EV6_LUT_FourWheel_EV6Battery77p4kWh_PowerCorrected/Vehicle Under Test1/Vehicle/Battery/Battery/Lithium Ion Battery Pack1/Datasheet Battery Internal ==
  BattCurr : Inport
  BattTemp : Inport  Port=2
  Constant1 : Constant  Value=BattCapInit
  Datasheet Battery : Subsystem  AncestorBlock=autolibbatterycommon/Datasheet Battery
  LdCurrFeed : Outport  VectorParamsAs1DForOutWhenUnconnected=off
  OutVoltUnfilt : Outport  Port=2  VectorParamsAs1DForOutWhenUnconnected=off
  LdAmpHr : Outport  Port=3  VectorParamsAs1DForOutWhenUnconnected=off
  BattSoc : Outport  Port=4  VectorParamsAs1DForOutWhenUnconnected=off
  BattPwrLoss : Outport  Port=5  VectorParamsAs1DForOutWhenUnconnected=off
  wires:
  Constant1/1 -> Datasheet Battery/1(CapInit)
  BattCurr/1 -> Datasheet Battery/2(BattCurr)
  BattTemp/1 -> Datasheet Battery/3(BattTemp)
  Datasheet Battery/4(BattSoc) -> BattSoc/1
  Datasheet Battery/3(LdAmpHr) -> LdAmpHr/1
  Datasheet Battery/2(OutVoltUnfilt) -> OutVoltUnfilt/1
  Datasheet Battery/1(LdCurrFeed) -> LdCurrFeed/1
  Datasheet Battery/5(BattPwrLoss) -> BattPwrLoss/1

== system EV6_LUT_FourWheel_EV6Battery77p4kWh_PowerCorrected/Vehicle Under Test1/Vehicle/Driver and Drive Cycle/Driver and PI with FF Control/Speed controller set/In-house CAVE ==
  note: BrakeSwitch
  RefSpd [km/hr] : Inport
  VehSpd : Inport  Port=2
  In-house Speed Controller : Subsystem
  AccelPedalCmd : Outport
  BrakePedalCmd : Outport  Port=2
  BrakeSwitch : Outport  Port=3
  wires:
  In-house Speed Controller/1(AcceleratorPedalPos) -> AccelPedalCmd/1  "AccelPedalCmd"
  VehSpd/1 -> In-house Speed Controller/2(VehicleSpeed)
  RefSpd [km/hr]/1 -> In-house Speed Controller/1(RefSpd)
  In-house Speed Controller/2(BrakePedalPos) -> BrakePedalCmd/1  "BrakePedalCmd"
  In-house Speed Controller/3(BrakeSwitch) -> BrakeSwitch/1

== system EV6_LUT_FourWheel_EV6Battery77p4kWh_PowerCorrected/Vehicle Under Test1/Vehicle/Driver and Drive Cycle/Driver and PI with FF Control/Speed controller set/PIF ==
  RefSpd [km/hr] : Inport
  VehSpd : Inport  Port=2
  Compare To Constant1 : simulink/Logic and Bit Operations/Compare To Constant  relop=<=  const=0.1  OutDataTypeStr=boolean  ZeroCross=off
  Constant : Constant  Value=0
  Constant1 : Constant  Value=0
  Gain : Gain  Gain=1/3.6
  Gain1 : Gain  Gain=1/3.6
  Gain2 : Gain  Gain=100
  Gain3 : Gain  Gain=100
  Longitudinal Driver : autolibshared/Longitudinal Driver  extAccelOvr=off  extDecelOvr=off  extAccelHld=off  extDecelHld=off  extAccelZero=off  extDecelZero=off  cntrlType=PI  shftType=None  velUnits=m/s  gearOut=off  Kp=2.5  Ki=1  Kff=.1*0.35  Kg=0  VehVelVec=[0 100]  KffVec=[.1 .1]  KpVec=[10 10]  KiVec=[5 5]  KgVec=[0 0]  m=1500  Kpt=3000  tau=.1  L=2  aR=200  bR=2.5  cR=.5  g=9.81  vnom=1  Kaw=1  tauerr=.01  tauPt=2  GearInit=0  tShift=.1  pdlVec=[0.1 0.4 0.5 0.9]  upShftTbl=[-1 12.9375 26.4375 39.9375 51.18749999999999 62.4375 72.84375 83.25;-1 16.3125 29.8125 43.3125 54.5624 65.8125 76.78125 87.75;-1 19.6875 33.1875 46.68749999999999 57.9375 69.1875 80.71875 92.25;-1 33 52.5 77.25 100.5 138.75 161.875 185]  dwnShftTbl=[1 9.5625 23.0625 36.5625 47.8125 59.0625 68.90625 78.75;1 12.9375 26.4375 39.9375 51.18749999999999 62.4375 72.84375 83.25;1 16.3125 29.8125 43.3125 54.562499 65.8125 76.78125 87.75;1 19.6875 33.1875 46.68749999999999 57.9375 69.1875 80.71875 92.25]  tClutch=.5  tRev=.5  tPark=120  aMode=2  UpGearVec="[0  1  2  3  4  5  6  7]"  DownGearVec="[1  2  3  4  5  6  7  8]"
      settings: LibrarySourceBlock=vehdynlibdriver/Longitudinal Driver
  Lowpass Filter : TransferFcn  Denominator=[.01 1]
  Min threshold for Brake switch : Constant  Value=0
  Relational Operator : RelationalOperator  Operator=>  OutDataTypeStr=boolean  InputSameDT=off
  Switch3 : Switch  Criteria=u2 > Threshold  SaturateOnIntegerOverflow=off  InputSameDT=off
  Switch4 : Switch  Criteria=u2 > Threshold  SaturateOnIntegerOverflow=off  InputSameDT=off
  Terminator : Terminator
  standstill brake [0,1] : Constant  Value=0.5
  AccelPedalCmd : Outport
  BrakePedalCmd : Outport  Port=2
  BrakeSwitch : Outport  Port=3
  wires:
  Lowpass Filter/1 -> Gain1/1  "VS_Flt"
  Switch4/1 -> Gain3/1  "BrakePedalPos_pct"
  Switch3/1 -> Gain2/1  "AcceleratorPedalPos_pct"
  standstill brake [0,1]/1 -> Switch4/1
  Compare To Constant1/1 -> Switch3/2, Switch4/2
  Constant/1 -> Switch3/1
  Longitudinal Driver/2 -> Switch3/3  "AcceleratorPedalPosPre_pct"
  Longitudinal Driver/1 -> Terminator/1
  Gain2/1 -> AccelPedalCmd/1  "AccelPedalCmd"
  Gain3/1 -> BrakePedalCmd/1  "BrakePedalCmd"
  VehSpd/1 -> Lowpass Filter/1
  RefSpd [km/hr]/1 -> Gain/1
  Constant1/1 -> Longitudinal Driver/3
  Gain/1 -> Longitudinal Driver/1, Compare To Constant1/1
  Longitudinal Driver/3 -> Relational Operator/1, Switch4/3  "BrakePedalPosPre_pct"
  Relational Operator/1 -> BrakeSwitch/1  "BrakeSwitch"
  Min threshold for Brake switch/1 -> Relational Operator/2
  Gain1/1 -> Longitudinal Driver/2

== system EV6_LUT_FourWheel_EV6Battery77p4kWh_PowerCorrected/Vehicle Under Test1/Vehicle/Driver and Drive Cycle/Driver and PI with FF Control/Speed controller set/Predictive ==
  RefSpd [km/hr] : Inport
  VehSpd : Inport  Port=2
  Compare To Constant1 : simulink/Logic and Bit Operations/Compare To Constant  relop=<=  const=0.1  OutDataTypeStr=boolean  ZeroCross=off
  Constant : Constant  Value=0
  Constant1 : Constant  Value=0
  Gain : Gain  Gain=1/3.6
  Gain1 : Gain  Gain=1/3.6
  Gain4 : Gain  Gain=100
  Gain5 : Gain  Gain=100
  Longitudinal Driver1 : Subsystem  Commented=on  Variant=on  VariantControlMode=label  VariantControl=Variant1  LabelModeActiveChoice=0  mask{tau=0.03, L=4, Kpt=10000}
      mask prompts: tau "Driver response time, tau [s]"; L "Preview distance, L [m]:"; Kpt "Effective vehicle total tractive force, Kpt [N]:"
      mask Display:
      | if strcmp('1',get_param(gcb,'ActiveVariant'))
      |     disp('Open Loop')
      | else
      |     image('LongitudinalDriver.png','center');
      | end
  Longitudinal Driver2 : autolibshared/Longitudinal Driver  extAccelOvr=off  extDecelOvr=off  extAccelHld=off  extDecelHld=off  extAccelZero=off  extDecelZero=off  cntrlType=Predictive  shftType=None  velUnits=m/s  gearOut=off  Kp=10  Ki=5  Kff=.1  Kg=0  VehVelVec=[0 100]  KffVec=[.1 .1]  KpVec=[10 10]  KiVec=[5 5]  KgVec=[0 0]  m=2040  Kpt=6500  tau=0.1  L=3  aR=200/10  bR=2.5/100  cR=.3  g=9.807  vnom=5  Kaw=1  tauerr=.01  tauPt=2  GearInit=0  tShift=.1  pdlVec=[0.1 0.4 0.5 0.9]  upShftTbl=[-1 12.9375 26.4375 39.9375 51.18749999999999 62.4375 72.84375 83.25;-1 16.3125 29.8125 43.3125 54.5624 65.8125 76.78125 87.75;-1 19.6875 33.1875 46.68749999999999 57.9375 69.1875 80.71875 92.25;-1 33 52.5 77.25 100.5 138.75 161.875 185]  dwnShftTbl=[1 9.5625 23.0625 36.5625 47.8125 59.0625 68.90625 78.75;1 12.9375 26.4375 39.9375 51.18749999999999 62.4375 72.84375 83.25;1 16.3125 29.8125 43.3125 54.562499 65.8125 76.78125 87.75;1 19.6875 33.1875 46.68749999999999 57.9375 69.1875 80.71875 92.25]  tClutch=.5  tRev=.5  tPark=120  aMode=2  UpGearVec="[0  1  2  3  4  5  6  7]"  DownGearVec="[1  2  3  4  5  6  7  8]"
      settings: LibrarySourceBlock=vehdynlibdriver/Longitudinal Driver
  Lowpass Filter : TransferFcn  Denominator=[.02 1]
  Min threshold for Brake switch : Constant  Value=0
  Relational Operator : RelationalOperator  Operator=>  OutDataTypeStr=boolean  InputSameDT=off
  Switch3 : Switch  Criteria=u2 > Threshold  SaturateOnIntegerOverflow=off  InputSameDT=off
  Switch4 : Switch  Criteria=u2 > Threshold  SaturateOnIntegerOverflow=off  InputSameDT=off
  Terminator : Terminator
  standstill brake [0,1] : Constant  Value=0.5
  AccelPedalCmd : Outport
  BrakePedalCmd : Outport  Port=2
  BrakeSwitch : Outport  Port=3
  wires:
  Lowpass Filter/1 -> Gain1/1  "VS_Flt"
  Longitudinal Driver2/2 -> Switch3/3  "AcceleratorPedalPosPre_pct"
  Gain5/1 -> BrakePedalCmd/1  "BrakePedalCmd"
  Gain/1 -> Longitudinal Driver2/1, Compare To Constant1/1
  Gain4/1 -> AccelPedalCmd/1  "AccelPedalCmd"
  Constant/1 -> Switch3/1
  Compare To Constant1/1 -> Switch3/2, Switch4/2
  Switch3/1 -> Gain4/1  "AcceleratorPedalPos_pct"
  Switch4/1 -> Gain5/1  "BrakePedalPos_pct"
  Longitudinal Driver2/3 -> Relational Operator/1, Switch4/3  "BrakePedalPosPre_pct"
  standstill brake [0,1]/1 -> Switch4/1
  Longitudinal Driver2/1 -> Terminator/1
  VehSpd/1 -> Lowpass Filter/1
  RefSpd [km/hr]/1 -> Gain/1
  Constant1/1 -> Longitudinal Driver2/3
  Relational Operator/1 -> BrakeSwitch/1  "BrakeSwitch"
  Min threshold for Brake switch/1 -> Relational Operator/2
  Gain1/1 -> Longitudinal Driver2/2

== system EV6_LUT_FourWheel_EV6Battery77p4kWh_PowerCorrected/Vehicle Under Test1/Vehicle/Driver and Drive Cycle/Driver and PI with FF Control/Speed controller set/Speed tracking controller ==
  RefSpd [km/hr] : Inport
  In2 : Inport  Port=2
  In-house CAVE : Subsystem  VariantControl=varaint1
  PIF : Subsystem  VariantControl=varaint2
  Predictive : Subsystem  VariantControl=varaint3
  AccelPedalCmd : Outport
  BrakePedalCmd : Outport  Port=2
  Out3 : Outport  Port=3

== system EV6_LUT_FourWheel_EV6Battery77p4kWh_PowerCorrected/Vehicle Under Test1/Vehicle/Powertrain Supervisory Controller /Engine Torque Command/Accel Pedal to Traction Wheel Torque Request1/Max Motor Torque ==
  MtrSpd : Inport
  Constant : Constant  Value=MtrPwrMax
  Divide : Product  Inputs=*/
  Saturation : Saturate  UpperLimit=MtrTrqMax  LowerLimit=0
  Saturation1 : Saturate  UpperLimit=inf  LowerLimit=1
  Scope : Scope
  Scope1 : Scope
  Scope2 : Scope
  MtrTrqMax : Outport
  wires:
  Constant/1 -> Divide/1
  MtrSpd/1 -> Scope2/1, Saturation1/1
  Divide/1 -> Scope1/1, Saturation/1
  Saturation1/1 -> Divide/2
  Saturation/1 -> Scope/1, MtrTrqMax/1

== system EV6_LUT_FourWheel_EV6Battery77p4kWh_PowerCorrected/Vehicle Under Test1/Vehicle/Powertrain Supervisory Controller /Engine Torque Command/EV6 Torque Distribution/Regen Brake Split LUT ==
  Accel_mps2 : Inport
  Speed_kph : Inport  Port=2
  MtrTrqCmd : Inport  Port=3
  Front Share 3D LUT : Lookup_n-D  NumberOfTableDimensions=3  BreakpointsForDimension1=accel_bp_mps2  BreakpointsForDimension2=speed_bp_kph  BreakpointsForDimension3=regen_torque_bp_Nm  Table=front_share_regen_3d  ExtrapMethod=Clip  InternalRulePriority=Speed  RndMeth=Simplest
      settings: InputPortMap=u0,u1,u2
  Front Torque Product : Product
  Limit Front Share : Saturate  UpperLimit=1  LowerLimit=0
  MotorToAxleTorque_LUT : Gain  Gain=EV6_FinalDriveRatio
  One : Constant
  Rear Share = 1 - Front : Sum  Inputs=+-
  Rear Torque Product : Product
  Torque Range : Saturate  UpperLimit=0  LowerLimit=-1400
  FrontShare : Outport
  RearShare : Outport  Port=2
  FrontMtrTrqCmd : Outport  Port=3
  RearMtrTrqCmd : Outport  Port=4
  wires:
  Accel_mps2/1 -> Front Share 3D LUT/1
  Speed_kph/1 -> Front Share 3D LUT/2
  MtrTrqCmd/1 -> MotorToAxleTorque_LUT/1, Front Torque Product/2, Rear Torque Product/2
  Torque Range/1 -> Front Share 3D LUT/3  "RegenAxleTorque_LUT_Input"
  Front Share 3D LUT/1 -> Limit Front Share/1
  Limit Front Share/1 -> Rear Share = 1 - Front/2, FrontShare/1, Front Torque Product/1
  One/1 -> Rear Share = 1 - Front/1
  Rear Share = 1 - Front/1 -> RearShare/1, Rear Torque Product/1
  Front Torque Product/1 -> FrontMtrTrqCmd/1
  Rear Torque Product/1 -> RearMtrTrqCmd/1
  MotorToAxleTorque_LUT/1 -> Torque Range/1  "RegenAxleTorque_PreSat"

== system EV6_LUT_FourWheel_EV6Battery77p4kWh_PowerCorrected/Vehicle Under Test1/Vehicle/Powertrain Supervisory Controller /Engine Torque Command/EV6 Torque Distribution/Traction Torque Split LUT ==
  Accel_mps2 : Inport
  Speed_kph : Inport  Port=2
  MtrTrqCmd : Inport  Port=3
  Front Share 3D LUT : Lookup_n-D  NumberOfTableDimensions=3  BreakpointsForDimension1=accel_bp_mps2  BreakpointsForDimension2=speed_bp_kph  BreakpointsForDimension3=traction_torque_bp_Nm  Table=front_share_traction_3d  ExtrapMethod=Clip  InternalRulePriority=Speed  RndMeth=Simplest
      settings: InputPortMap=u0,u1,u2
  Front Torque Product : Product
  Limit Front Share : Saturate  UpperLimit=1  LowerLimit=0
  MotorToAxleTorque_LUT : Gain  Gain=EV6_FinalDriveRatio
  One : Constant
  Rear Share = 1 - Front : Sum  Inputs=+-
  Rear Torque Product : Product
  Torque Range : Saturate  UpperLimit=1300  LowerLimit=0
  FrontShare : Outport
  RearShare : Outport  Port=2
  FrontMtrTrqCmd : Outport  Port=3
  RearMtrTrqCmd : Outport  Port=4
  wires:
  Accel_mps2/1 -> Front Share 3D LUT/1
  Speed_kph/1 -> Front Share 3D LUT/2
  MtrTrqCmd/1 -> MotorToAxleTorque_LUT/1, Front Torque Product/2, Rear Torque Product/2
  Torque Range/1 -> Front Share 3D LUT/3  "TractionAxleTorque_LUT_Input"
  Front Share 3D LUT/1 -> Limit Front Share/1
  Limit Front Share/1 -> FrontShare/1, Front Torque Product/1, Rear Share = 1 - Front/2
  One/1 -> Rear Share = 1 - Front/1
  Rear Share = 1 - Front/1 -> RearShare/1, Rear Torque Product/1
  Front Torque Product/1 -> FrontMtrTrqCmd/1
  Rear Torque Product/1 -> RearMtrTrqCmd/1
  MotorToAxleTorque_LUT/1 -> Torque Range/1  "TractionAxleTorque_PreSat"
